simulink model "CalibAdc"  (R2023b)
settings: Solver=FixedStepDiscrete  StartTime=0.0  StopTime=10.0  FixedStep=1e-4  RelTol=1e-3
undefined symbols (not defined in the file): CALIBADC_BIAS_I_ADC_TO_CURR, CALIBADC_BIAS_V_ADC_TO_VOLT, CALIBADC_GAIN_I_ADC_TO_CURR, CALIBADC_GAIN_V_ADC_TO_VOLT
settings Model: DataDictionary=CalibAdc.sldd  Creator=84339  LastModifiedBy=84339
settings OptimizationCC: DefaultParameterBehavior=Inlined  EnhancedBackFolding=on  PassReuseOutputArgsAs=Individual arguments  ZeroExternalMemoryAtStartup=off  ZeroInternalMemoryAtStartup=off  OptimizeBlockOrder=speed  DifferentSizesBufferReuse=on  OptimizationCustomize=off  EfficientTunableParamExpr=on
settings DebuggingCC: ParameterTunabilityLossMsg=error
settings SFSimCC: MATLABDynamicMemAlloc=off
settings RTWCC: Description=Embedded Coder  SystemTargetFile=ert.tlc  EmbeddedCoderDictionary=Arch.sldd  GenCodeOnly=on  TemplateMakefile=ert_default_tmf
settings CodeAppCC: ForceParamTrailComments=on  IgnoreCustomStorageClasses=off  OperatorAnnotations=on  SimulinkDataObjDesc=on  SFDataObjDesc=on  InsertBlockDesc=on
settings ERTTargetCC: TargetLangStandard=C99 (ISO)  GenerateSampleERTMain=on  InlinedParameterPlacement=NonHierarchical  ERTCustomFileTemplate=example_file_process.tlc

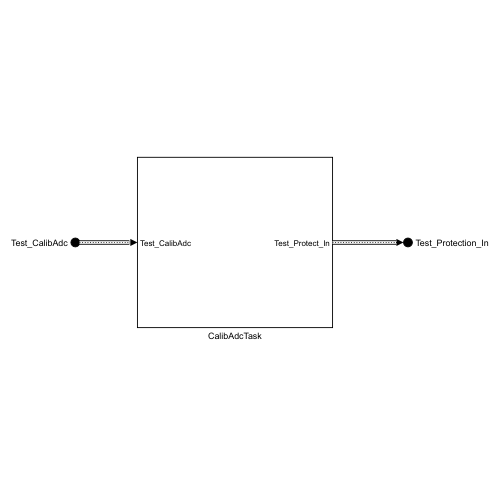
[thumbnail: Simulink's stored preview of the top-level diagram]
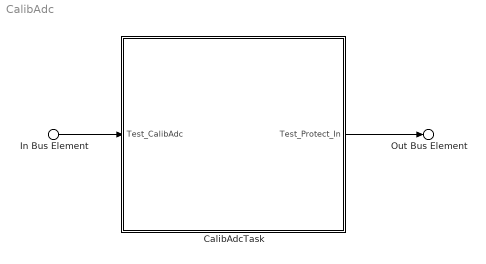
== system CalibAdc ==
  In Bus Element : Inport  PortName=Test_CalibAdc
  CalibAdcTask : Subsystem
  Out Bus Element : Outport  PortName=Test_Protection_In
  wires:
  In Bus Element/1 -> CalibAdcTask/1(Test_CalibAdc)
  CalibAdcTask/1(Test_Protect_In) -> Out Bus Element/1

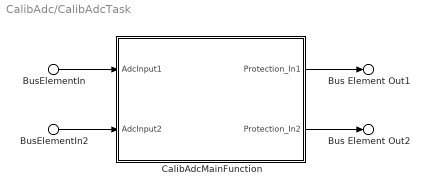
== system CalibAdc/CalibAdcTask ==
  BusElementIn : Inport  PortName=Test_CalibAdc  Element=AdcInput1
  BusElementIn2 : Inport  PortName=Test_CalibAdc  Element=AdcInput2
  CalibAdcMainFunction : Subsystem
  Bus Element Out1 : Outport  PortName=Test_Protect_In  Element=Protection_In1
  Bus Element Out2 : Outport  PortName=Test_Protect_In  Element=Protection_In2
  wires:
  BusElementIn/1 -> CalibAdcMainFunction/1(AdcInput1)
  BusElementIn2/1 -> CalibAdcMainFunction/2(AdcInput2)
  CalibAdcMainFunction/1(Protection_In1) -> Bus Element Out1/1
  CalibAdcMainFunction/2(Protection_In2) -> Bus Element Out2/1

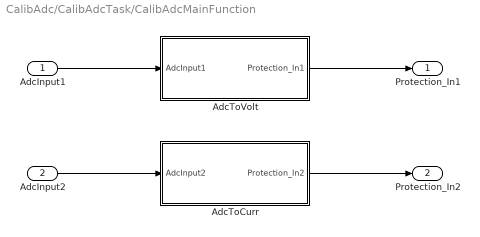
== system CalibAdc/CalibAdcTask/CalibAdcMainFunction ==
  AdcInput1 : Inport
  AdcInput2 : Inport  Port=2
  AdcToCurr : Subsystem
  AdcToVolt : Subsystem
  Protection_In1 : Outport
  Protection_In2 : Outport  Port=2
  wires:
  AdcToVolt/1(Protection_In1) -> Protection_In1/1
  AdcInput2/1 -> AdcToCurr/1(AdcInput2)
  AdcToCurr/1(Protection_In2) -> Protection_In2/1
  AdcInput1/1 -> AdcToVolt/1(AdcInput1)

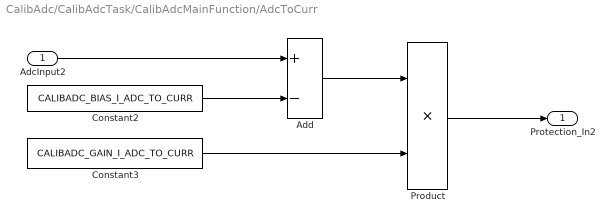
== system CalibAdc/CalibAdcTask/CalibAdcMainFunction/AdcToCurr ==
  AdcInput2 : Inport
  Add : Sum  Inputs=+-
  Constant2 : Constant  Value=CALIBADC_BIAS_I_ADC_TO_CURR  OutDataTypeStr=single  SampleTime=-1
  Constant3 : Constant  Value=CALIBADC_GAIN_I_ADC_TO_CURR  OutDataTypeStr=single  SampleTime=-1
  Product : Product
  Protection_In2 : Outport
  wires:
  AdcInput2/1 -> Add/1
  Add/1 -> Product/1
  Constant3/1 -> Product/2
  Constant2/1 -> Add/2
  Product/1 -> Protection_In2/1

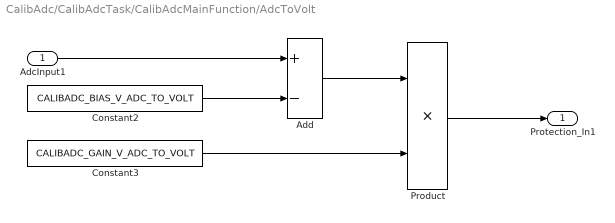
== system CalibAdc/CalibAdcTask/CalibAdcMainFunction/AdcToVolt ==
  AdcInput1 : Inport
  Add : Sum  Inputs=+-
  Constant2 : Constant  Value=CALIBADC_BIAS_V_ADC_TO_VOLT  OutDataTypeStr=single  SampleTime=-1
  Constant3 : Constant  Value=CALIBADC_GAIN_V_ADC_TO_VOLT  OutDataTypeStr=single  SampleTime=-1
  Product : Product
  Protection_In1 : Outport
  wires:
  AdcInput1/1 -> Add/1
  Add/1 -> Product/1
  Constant3/1 -> Product/2
  Constant2/1 -> Add/2
  Product/1 -> Protection_In1/1
